simulink model "cooling_loop"  (R2026b)
settings: Solver=ode4  StartTime=0  StopTime=1726  FixedStep=0.10000000000000001
model workspace (MAT data in the model file):
  C = 30000
  T0 = 85
  T_amb = 31
  cyc_Qin = [2000 2000 2000 2000 2000 2000 2000 2000 2000 2000 2000 2000 ... (17261 elements, 1x17261)]
  cyc_mdot = [2.23596170404 2.23596170404 2.23596170404 2.23596170404 2.23596170404 2.23596170404 2.23596170404 2.23596170404 2.23596170404 2.23596170404 2.23596170404 2.23596170404 ... (17261 elements, 1x17261)]
  cyc_t = [0 0.1 0.2 0.3 0.4 0.5 0.6 0.7 0.8 0.9 1 1.1 ... (17261 elements, 1x17261)]
  cyc_v = [0 0 0 0 0 0 0 0 0 0 0 0 ... (17261 elements, 1x17261)]
  dt = 0.1
  eta_ram = 0.3
  fan_cfm = 300
  fan_off = 90
  fan_on = 95
  hA_ext = 10
  thermo_full = 95
  thermo_min = 0.02
  thermo_open = 82
(part 1 of 2)
settings Model: Creator=admin  LastModifiedBy=admin

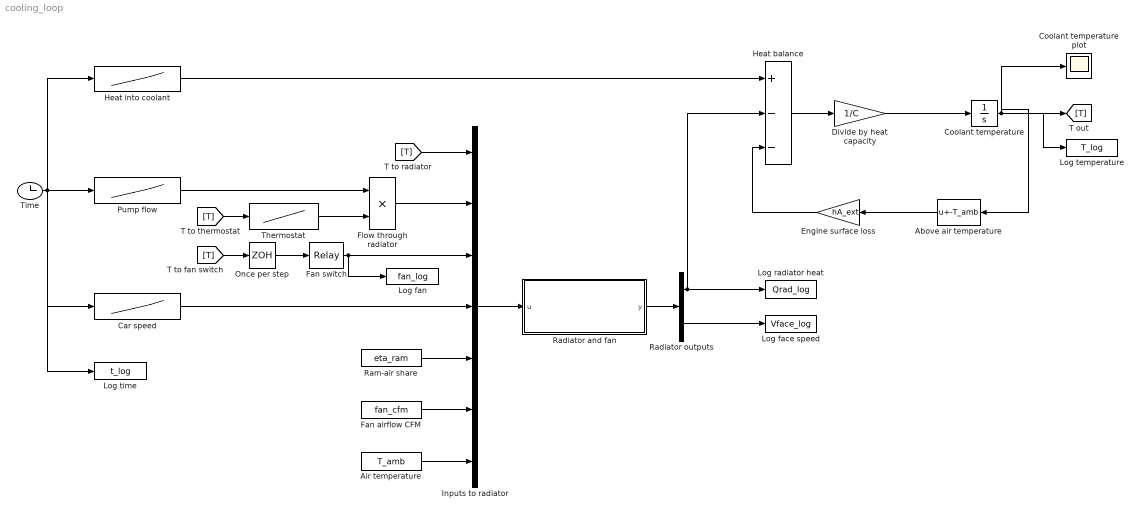
== system cooling_loop ==
  Above air temperature : Bias  Bias=-T_amb  SaturateOnIntegerOverflow=off
  Air temperature : Constant  Value=T_amb
  Car speed : Lookup_n-D  NumberOfTableDimensions=1  BreakpointsForDimension1=cyc_t  Table=cyc_v  ExtrapMethod=Clip  InternalRulePriority=Speed  RndMeth=Simplest
  Coolant temperature : Integrator  InitialCondition=T0
  Coolant temperature plot : Scope
  Divide by heat capacity : Gain  Gain=1/C
  Engine surface loss : Gain  Gain=hA_ext
  Fan airflow CFM : Constant  Value=fan_cfm
  Fan switch : Relay  OnSwitchValue=fan_on  OffSwitchValue=fan_off
  Flow through radiator : Product
  Heat balance : Sum  Inputs=+--
  Heat into coolant : Lookup_n-D  NumberOfTableDimensions=1  BreakpointsForDimension1=cyc_t  Table=cyc_Qin  ExtrapMethod=Clip  InternalRulePriority=Speed  RndMeth=Simplest
  Inputs to radiator : Mux  Inputs=7
  Log face speed : ToWorkspace  VariableName=Vface_log  SampleTime=dt
  Log fan : ToWorkspace  VariableName=fan_log  SampleTime=dt
  Log radiator heat : ToWorkspace  VariableName=Qrad_log  SampleTime=dt
  Log temperature : ToWorkspace  VariableName=T_log  SampleTime=dt
  Log time : ToWorkspace  VariableName=t_log  SampleTime=dt
  Once per step : ZeroOrderHold  SampleTime=dt
  Pump flow : Lookup_n-D  NumberOfTableDimensions=1  BreakpointsForDimension1=cyc_t  Table=cyc_mdot  ExtrapMethod=Clip  InternalRulePriority=Speed  RndMeth=Simplest
  Radiator and fan : MATLAB Function  TreatAsAtomicUnit=on
  Radiator outputs : Demux  Outputs=2
  Ram-air share : Constant  Value=eta_ram
  Thermostat : Lookup_n-D  NumberOfTableDimensions=1  BreakpointsForDimension1=[thermo_open thermo_full]  Table=[thermo_min 1]  ExtrapMethod=Clip  InternalRulePriority=Speed  RndMeth=Simplest
  Time : Clock
  wires:
  Time/1 -> Pump flow/1, Heat into coolant/1, Car speed/1, Log time/1
  [T] -> Thermostat/1
  Pump flow/1 -> Flow through radiator/1
  Thermostat/1 -> Flow through radiator/2
  [T] -> Once per step/1
  Once per step/1 -> Fan switch/1
  [T] -> Inputs to radiator/1
  Flow through radiator/1 -> Inputs to radiator/2
  Fan switch/1 -> Inputs to radiator/3, Log fan/1
  Car speed/1 -> Inputs to radiator/4
  Ram-air share/1 -> Inputs to radiator/5
  Fan airflow CFM/1 -> Inputs to radiator/6
  Air temperature/1 -> Inputs to radiator/7
  Inputs to radiator/1 -> Radiator and fan/1(u)
  Radiator and fan/1(y) -> Radiator outputs/1
  Radiator outputs/1 -> Log radiator heat/1, Heat balance/2
  Radiator outputs/2 -> Log face speed/1
  Heat into coolant/1 -> Heat balance/1
  Heat balance/1 -> Divide by heat capacity/1
  Divide by heat capacity/1 -> Coolant temperature/1
  Coolant temperature/1 -> [T], Coolant temperature plot/1, Log temperature/1, Above air temperature/1
  Above air temperature/1 -> Engine surface loss/1
  Engine surface loss/1 -> Heat balance/3
